simulink model "W06_8_ned"  (R2024b)
settings: Solver=ode4  StartTime=0.0  StopTime=T_run  FixedStep=Ts_ctrl  RelTol=1e-3
InitFcn:
  | if ~exist('W06_model_init','file'), addpath(fileparts(get_param('W06_8_ned','FileName'))); end, W06_model_init('W06_8_ned')
StopFcn:
  | W06_model_done('W06_8_ned')
values from neighbouring files (symbols this model uses):
  alloc_prm = [half_beam; l_bow; F_max; F_bow_max]    [W06_setup.m]
  animate = 0    [W06_bow_demo.m]    (also in W06_psi_sweep.m; W06_setup.m = 1)
  beta_c = deg2rad(current_direction)    [W06_setup.m]
  bow_on = BOW(i)    [W06_bow_demo.m]    (also in W06_setup.m = 1)
  current_speed = 0.0    (= 0)    [W06_setup.m]
  F_bow_max = 250    [W06_setup.m]
  F_max = 500    [W06_setup.m]
  F_plugin_max = 2353.53383667818    (= 2353.53383668)    [W06_setup.m]
  half_beam = 1.027135    [W06_setup.m]
  k_prop = 1000 * 0.004422 * 0.2^4    (= 0.0070752)    [W06_setup.m]
  Kb = Ki_u / Kp_u    (= 0.333333333333)    [W06_setup.m]
  Kd_psi = 200    [W06_setup.m]
  Ki_vn = 100    [W06_setup.m]
  Kp_ned = 0.4    [W06_setup.m]
  Kp_psi = 400    [W06_setup.m]
  Kp_vn = 300    [W06_setup.m]
  l_bow = 0.75    [W06_setup.m]
  stop_hold = 15    [W06_setup.m]
  task_mode = 3    [W06_setup.m]
  task_q = [ hold_north;  hold_east;  deg2rad(hold_deg) ... (first row only)    [W06_setup.m]
  Ts_ctrl = 0.05    [W06_setup.m]
  usv_p = [m_usv; Izz; Xu; Xuu; Yv; Yvv; Nr; Nrr; half_beam; l_bow]    [W06_setup.m]
  V_ned_max = v_max    (= 0.6)    [W06_setup.m]
  x0 = [0.1; 0; 0; 0; 0; psi_init]    [W06_setup.m]
libraries: slpidlib x2
settings Model: Creator=admin  LastModifiedBy=admin

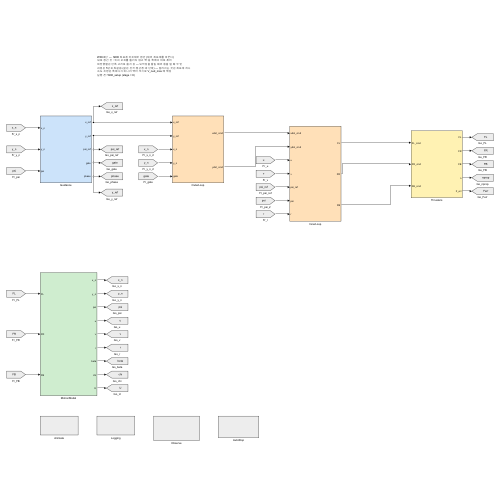
[thumbnail: Simulink's stored preview of the top-level diagram]
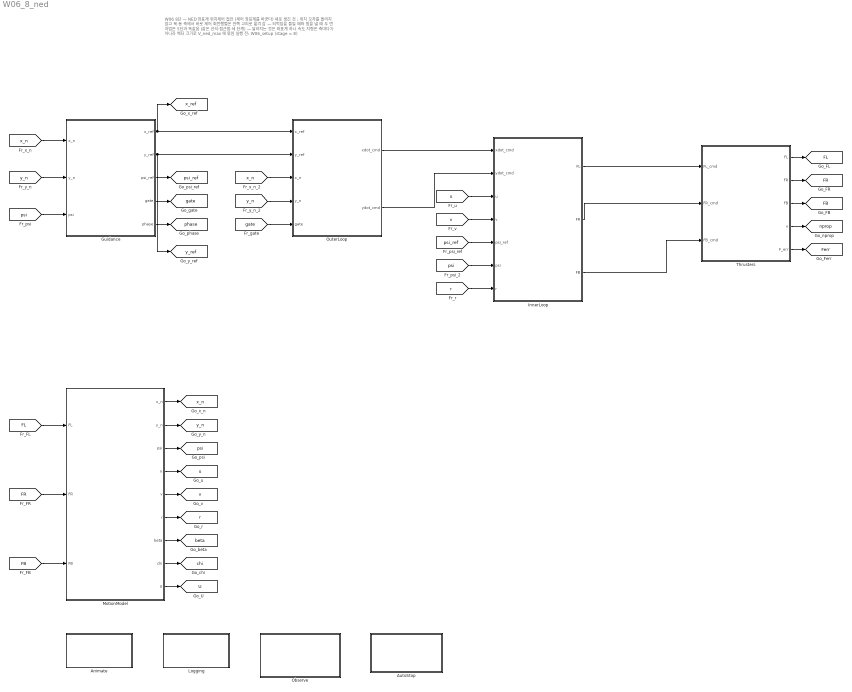
== system W06_8_ned ==
  note: W06 8단  —  NED 좌표계 위치제어 접안 (제어 좌표계를 바꾼다)
      | 새로 생긴 것 : 위치 오차를 돌리지 않고 북·동 축에서 바로 제어
      | 회전행렬은 안쪽 고리로 옮겨 감 — 되먹임을 들일 때와 힘을 낼 때 두 번
      | 과업은 5단과 똑같음 (같은 선석·접근점·세 단계) — 달라지는 것은 좌표계 하나
      | 속도 지령은 축마다가 아니라 벡터 크기로 V_ned_max 에 묶임
      | 실행 전: W06_setup (stage = 8)
  Animate : Subsystem
  AutoStop : Subsystem
  Guidance : Subsystem
  InnerLoop : Subsystem
  Logging : Subsystem
  MotionModel : Subsystem
  Observe : Subsystem
  OuterLoop : Subsystem
  Thrusters : Subsystem
  tag scope: FB=global, FL=global, FR=global, Ferr=global, U=global, beta=global, chi=global, gate=global, nprop=global, phase=global, psi=global, psi_ref=global, r=global, u=global, v=global, x_n=global, x_ref=global, y_n=global, y_ref=global
  wires:
  InnerLoop/3(FB) -> Thrusters/3(FB_cmd)
  InnerLoop/2(FR) -> Thrusters/2(FR_cmd)
  InnerLoop/1(FL) -> Thrusters/1(FL_cmd)
  OuterLoop/2(ydot_cmd) -> InnerLoop/2(ydot_cmd)
  OuterLoop/1(xdot_cmd) -> InnerLoop/1(xdot_cmd)
  Guidance/1(x_ref) -> OuterLoop/1(x_ref), [x_ref]
  Guidance/2(y_ref) -> OuterLoop/2(y_ref), [y_ref]
  Thrusters/1(FL) -> [FL]
  Thrusters/2(FR) -> [FR]
  Thrusters/4(n) -> [nprop]
  MotionModel/3(psi) -> [psi]
  Guidance/3(psi_ref) -> [psi_ref]
  MotionModel/6(r) -> [r]
  MotionModel/4(u) -> [u]
  MotionModel/5(v) -> [v]
  MotionModel/1(x_n) -> [x_n]
  MotionModel/2(y_n) -> [y_n]
  [FB] -> MotionModel/3(FB)
  [FL] -> MotionModel/1(FL)
  [FR] -> MotionModel/2(FR)
  [psi_ref] -> InnerLoop/5(psi_ref)
  [r] -> InnerLoop/7(r)
  [v] -> InnerLoop/4(v)
  [x_n] -> Guidance/1(x_n)
  [x_n] -> OuterLoop/3(x_n)
  [y_n] -> Guidance/2(y_n)
  [y_n] -> OuterLoop/4(y_n)
  Thrusters/3(FB) -> [FB]
  Thrusters/5(F_err) -> [Ferr]
  MotionModel/9(U) -> [U]
  MotionModel/7(beta) -> [beta]
  MotionModel/8(chi) -> [chi]
  Guidance/4(gate) -> [gate]
  Guidance/5(phase) -> [phase]
  [gate] -> OuterLoop/5(gate)
  [psi] -> Guidance/3(psi)
  [psi] -> InnerLoop/6(psi)
  [u] -> InnerLoop/3(u)

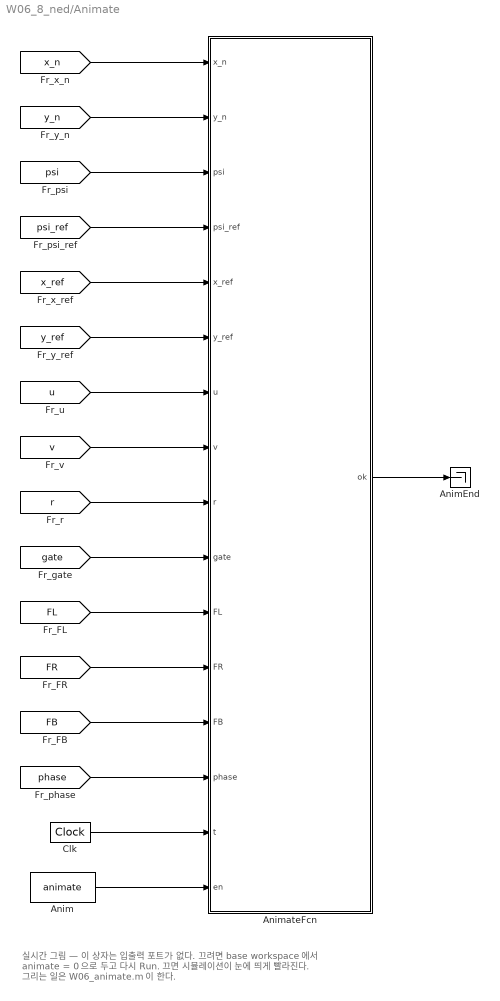
== system W06_8_ned/Animate ==
  note: 실시간 그림 — 이 상자는 입출력 포트가 없다.
      | 끄려면 base workspace 에서  animate = 0  으로 두고 다시 Run.
      | 끄면 시뮬레이션이 눈에 띄게 빨라진다.
      | 그리는 일은 W06_animate.m 이 한다.
  Anim : Constant  Value=animate
  AnimEnd : Terminator
  AnimateFcn : MATLAB Function  TreatAsAtomicUnit=on
  Clk : DigitalClock  SampleTime=Ts_ctrl
  wires:
  [x_n] -> AnimateFcn/1(x_n)
  [y_n] -> AnimateFcn/2(y_n)
  [psi] -> AnimateFcn/3(psi)
  [psi_ref] -> AnimateFcn/4(psi_ref)
  [x_ref] -> AnimateFcn/5(x_ref)
  [y_ref] -> AnimateFcn/6(y_ref)
  [u] -> AnimateFcn/7(u)
  [v] -> AnimateFcn/8(v)
  [r] -> AnimateFcn/9(r)
  [gate] -> AnimateFcn/10(gate)
  [FL] -> AnimateFcn/11(FL)
  [FR] -> AnimateFcn/12(FR)
  [FB] -> AnimateFcn/13(FB)
  [phase] -> AnimateFcn/14(phase)
  Clk/1 -> AnimateFcn/15(t)
  Anim/1 -> AnimateFcn/16(en)
  AnimateFcn/1(ok) -> AnimEnd/1

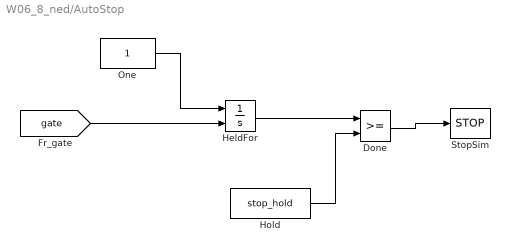
== system W06_8_ned/AutoStop ==
  Done : RelationalOperator  OutDataTypeStr=boolean  RndMeth=Simplest  InputSameDT=off
  HeldFor : Integrator  ExternalReset=level
  Hold : Constant  Value=stop_hold
  One : Constant
  StopSim : Stop
  wires:
  One/1 -> HeldFor/1
  [gate] -> HeldFor/2
  HeldFor/1 -> Done/1
  Hold/1 -> Done/2
  Done/1 -> StopSim/1

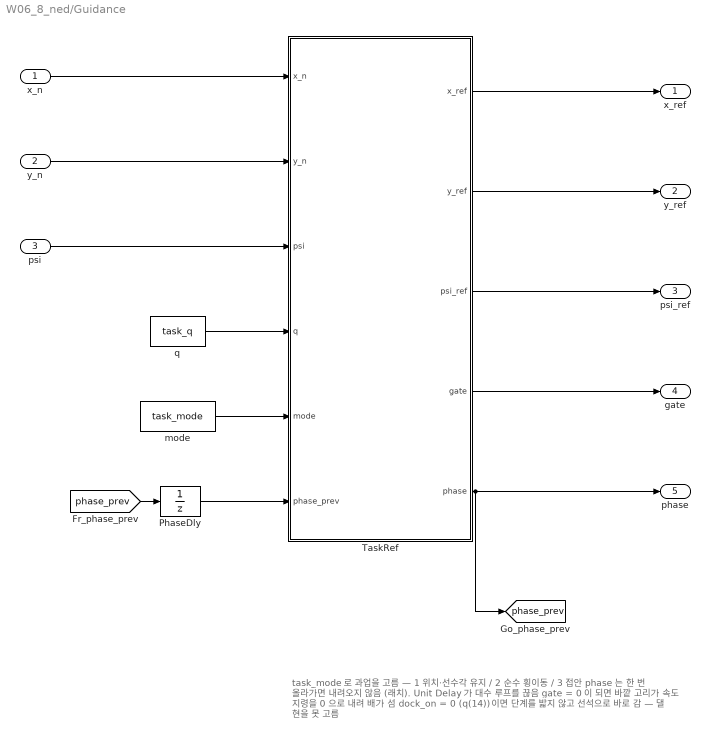
== system W06_8_ned/Guidance ==
  note: task_mode 로 과업을 고름 — 1 위치·선수각 유지 / 2 순수 횡이동 / 3 접안
      | phase 는 한 번 올라가면 내려오지 않음 (래치). Unit Delay 가 대수 루프를 끊음
      | gate = 0 이 되면 바깥 고리가 속도 지령을 0 으로 내려 배가 섬
      | dock_on = 0 (q(14)) 이면 단계를 밟지 않고 선석으로 바로 감 — 댈 현을 못 고름
  x_n : Inport
  y_n : Inport  Port=2
  psi : Inport  Port=3
  PhaseDly : UnitDelay  Description=phase 래치가 자기 자신을 입력으로 받으므로 그대로 되먹이면 대수 루프가 된다. 한 스텝 전 값을 쓰는 것 말고는 끊을 방법이 없는 자리다. 표본 간격을 고정 스텝(Ts_ctrl)과 같게 두어 연속 솔버(ode4)와 어긋나지 않는다.  SampleTime=Ts_ctrl  HasFrameUpgradeWarning=on
  TaskRef : MATLAB Function  TreatAsAtomicUnit=on
  mode : Constant  Value=task_mode
  q : Constant  Value=task_q
  x_ref : Outport
  y_ref : Outport  Port=2
  psi_ref : Outport  Port=3
  gate : Outport  Port=4
  phase : Outport  Port=5
  tag scope: phase_prev=global
  wires:
  x_n/1 -> TaskRef/1(x_n)
  y_n/1 -> TaskRef/2(y_n)
  psi/1 -> TaskRef/3(psi)
  q/1 -> TaskRef/4(q)
  mode/1 -> TaskRef/5(mode)
  PhaseDly/1 -> TaskRef/6(phase_prev)
  TaskRef/1(x_ref) -> x_ref/1
  TaskRef/2(y_ref) -> y_ref/1
  TaskRef/3(psi_ref) -> psi_ref/1
  TaskRef/4(gate) -> gate/1
  TaskRef/5(phase) -> phase/1, [phase_prev]
  [phase_prev] -> PhaseDly/1

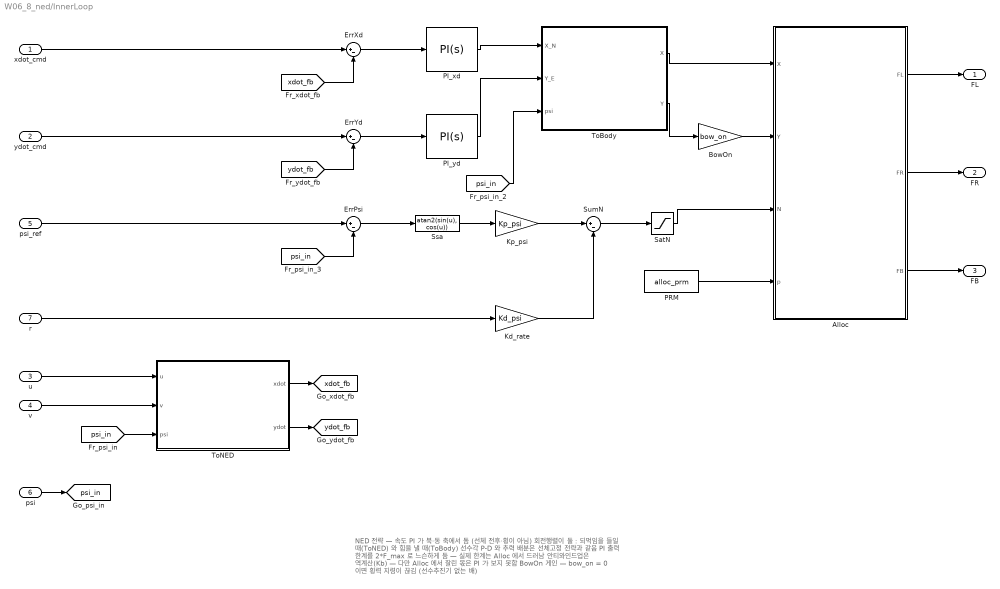
== system W06_8_ned/InnerLoop ==
  note: NED 전략 — 속도 PI 가 북·동 축에서 돔 (선체 전후·횡이 아님)
      | 회전행렬이 둘 : 되먹임을 들일 때(ToNED) 와 힘을 낼 때(ToBody)
      | 선수각 P-D 와 추력 배분은 선체고정 전략과 같음
      | PI 출력 한계를 2*F_max 로 느슨하게 둠 — 실제 한계는 Alloc 에서 드러남
      | 안티와인드업은 역계산(Kb) — 다만 Alloc 에서 잘린 몫은 PI 가 보지 못함
      | BowOn 게인 — bow_on = 0 이면 횡력 지령이 끊김 (선수추진기 없는 배)
  xdot_cmd : Inport
  ydot_cmd : Inport  Port=2
  u : Inport  Port=3
  v : Inport  Port=4
  psi_ref : Inport  Port=5
  psi : Inport  Port=6
  r : Inport  Port=7
  Alloc : MATLAB Function  TreatAsAtomicUnit=on
  BowOn : Gain  Gain=bow_on
  ErrPsi : Sum  Inputs=|+-
  ErrXd : Sum  Inputs=|+-
  ErrYd : Sum  Inputs=|+-
  Kd_rate : Gain  Gain=Kd_psi
  Kp_psi : Gain  Gain=Kp_psi
  PI_xd : slpidlib/PID Controller  Controller=PI  Form=Parallel  TimeDomain=Continuous-time  UseExternalTs=off  SampleTime=-1  IntegratorMethod=Forward Euler  FilterMethod=Forward Euler  ControllerParametersSource=internal  P=Kp_vn  I=Ki_vn  UseKiTs=off  D=0  UseExternalDerivativeSource=off  N=100  UseFilter=on  TunerSelectOption=Transfer Function Based (PID Tuner App)  InitialConditionSource=internal  InitialConditionForIntegrator=0  InitialConditionForFilter=0  DifferentiatorICPrevScaledInput=0  ExternalReset=none  TrackingMode=off  Kt=1  LimitOutput=on  SatLimitsSource=internal  UpperSaturationLimit=2*F_max  LowerSaturationLimit=-(2*F_max)  LinearizeAsGain=on  AntiWindupMode=back-calculation  Kb=Kb  LimitIntegrator=off  UpperIntegratorSaturationLimit=inf  LowerIntegratorSaturationLimit=-inf  POutMin=[]  POutMax=[]  IOutMin=[]  IOutMax=[]  DOutMin=[]  DOutMax=[]  NOutMin=[]  NOutMax=[]  SumOutMin=[]  SumOutMax=[]  SaturationOutMin=[]  SaturationOutMax=[]  PParamMin=[]  PParamMax=[]  IParamMin=[]  IParamMax=[]  DParamMin=[]  DParamMax=[]  NParamMin=[]  NParamMax=[]  KbParamMin=[]  KbParamMax=[]  KtParamMin=[]  KtParamMax=[]  KbOutMin=[]  KbOutMax=[]  KtOutMin=[]  KtOutMax=[]  IntegratorOutMin=[]  IntegratorOutMax=[]  FilterOutMin=[]  FilterOutMax=[]  SumI1OutMin=[]  SumI1OutMax=[]  SumI2OutMin=[]  SumI2OutMax=[]  SumI3OutMin=[]  SumI3OutMax=[]  SumI4OutMin=[]  SumI4OutMax=[]  SumDOutMin=[]  SumDOutMax=[]  DifferentiatorOutMin=[]  DifferentiatorOutMax=[]  FilterDiffOutCoefMin=[]  FilterDiffOutCoefMax=[]  ReciprocalOutMin=[]  ReciprocalOutMax=[]  SumDenOutMin=[]  SumDenOutMax=[]  SumNumOutMin=[]  SumNumOutMax=[]  DivideOutMin=[]  DivideOutMax=[]  UdiffTsProdOutMin=[]  UdiffTsProdOutMax=[]  NTsProdOutMin=[]  NTsProdOutMax=[]  UintegralTsProdOutMin=[]  UintegralTsProdOutMax=[]  UngainTsProdOutMin=[]  UngainTsProdOutMax=[]  ClampingZeroOutDataTypeStr=Inherit: Inherit via back propagation  ClampingZeroOutMin=[]  ClampingZeroOutMax=[]  FilterDenConstantOutDataTypeStr=Inherit: Inherit via back propagation  FilterDenConstantOutMin=[]  FilterDenConstantOutMax=[]  PCopyOutDataTypeStr=Inherit: Inherit via back propagation  PCopyOutMin=[]  PCopyOutMax=[]  NCopyOutDataTypeStr=Inherit: Inherit via back propagation  NCopyOutMin=[]  NCopyOutMax=[]  IntegratorContinuousStateAttributes=''  IntegratorStateMustResolveToSignalObject=off  IntegratorRTWStateStorageClass=Auto  FilterContinuousStateAttributes=''  FilterStateMustResolveToSignalObject=off  FilterRTWStateStorageClass=Auto  ParallelPVariant=InternalParameters  IdealPVariant=Disabled  IVariant=InternalParameters  DVariant=Disabled  IntegratorVariant=Continuous  SatVariant=Enabled  AWVariant=BackCalculation  PCopyVariant=Disabled  TRVariant=Disabled  FdbkBlocksVariant=Forward  IdealPFdbkVariant=Disabled  SatFdbkVariant=Disabled  DerivativeFilterVariant=Disabled  NVariant=Disabled  NCopyVariant=Disabled_SignalSpec  FilterICVariant=Disabled  IntegratorICVariant=InternalICs  ExternalResetVariant=Disabled  TRSumVariant=Passthrough  SumFdbkVariant=Disabled  SumVariant=Sum_PI  TsampFilterVariant=InternalTs  TsampNgainVariant=Passthrough  TsampIntegralVariant=Disabled_SignalSpec  ExternalSaturationOutDataTypeStr=Inherit: Same as second input  DerivativeSourceVariant=Disabled  PreIntVariant=InternalPreInt
  PI_yd : slpidlib/PID Controller  Controller=PI  Form=Parallel  TimeDomain=Continuous-time  UseExternalTs=off  SampleTime=-1  IntegratorMethod=Forward Euler  FilterMethod=Forward Euler  ControllerParametersSource=internal  P=Kp_vn  I=Ki_vn  UseKiTs=off  D=0  UseExternalDerivativeSource=off  N=100  UseFilter=on  TunerSelectOption=Transfer Function Based (PID Tuner App)  InitialConditionSource=internal  InitialConditionForIntegrator=0  InitialConditionForFilter=0  DifferentiatorICPrevScaledInput=0  ExternalReset=none  TrackingMode=off  Kt=1  LimitOutput=on  SatLimitsSource=internal  UpperSaturationLimit=2*F_max  LowerSaturationLimit=-(2*F_max)  LinearizeAsGain=on  AntiWindupMode=back-calculation  Kb=Kb  LimitIntegrator=off  UpperIntegratorSaturationLimit=inf  LowerIntegratorSaturationLimit=-inf  POutMin=[]  POutMax=[]  IOutMin=[]  IOutMax=[]  DOutMin=[]  DOutMax=[]  NOutMin=[]  NOutMax=[]  SumOutMin=[]  SumOutMax=[]  SaturationOutMin=[]  SaturationOutMax=[]  PParamMin=[]  PParamMax=[]  IParamMin=[]  IParamMax=[]  DParamMin=[]  DParamMax=[]  NParamMin=[]  NParamMax=[]  KbParamMin=[]  KbParamMax=[]  KtParamMin=[]  KtParamMax=[]  KbOutMin=[]  KbOutMax=[]  KtOutMin=[]  KtOutMax=[]  IntegratorOutMin=[]  IntegratorOutMax=[]  FilterOutMin=[]  FilterOutMax=[]  SumI1OutMin=[]  SumI1OutMax=[]  SumI2OutMin=[]  SumI2OutMax=[]  SumI3OutMin=[]  SumI3OutMax=[]  SumI4OutMin=[]  SumI4OutMax=[]  SumDOutMin=[]  SumDOutMax=[]  DifferentiatorOutMin=[]  DifferentiatorOutMax=[]  FilterDiffOutCoefMin=[]  FilterDiffOutCoefMax=[]  ReciprocalOutMin=[]  ReciprocalOutMax=[]  SumDenOutMin=[]  SumDenOutMax=[]  SumNumOutMin=[]  SumNumOutMax=[]  DivideOutMin=[]  DivideOutMax=[]  UdiffTsProdOutMin=[]  UdiffTsProdOutMax=[]  NTsProdOutMin=[]  NTsProdOutMax=[]  UintegralTsProdOutMin=[]  UintegralTsProdOutMax=[]  UngainTsProdOutMin=[]  UngainTsProdOutMax=[]  ClampingZeroOutDataTypeStr=Inherit: Inherit via back propagation  ClampingZeroOutMin=[]  ClampingZeroOutMax=[]  FilterDenConstantOutDataTypeStr=Inherit: Inherit via back propagation  FilterDenConstantOutMin=[]  FilterDenConstantOutMax=[]  PCopyOutDataTypeStr=Inherit: Inherit via back propagation  PCopyOutMin=[]  PCopyOutMax=[]  NCopyOutDataTypeStr=Inherit: Inherit via back propagation  NCopyOutMin=[]  NCopyOutMax=[]  IntegratorContinuousStateAttributes=''  IntegratorStateMustResolveToSignalObject=off  IntegratorRTWStateStorageClass=Auto  FilterContinuousStateAttributes=''  FilterStateMustResolveToSignalObject=off  FilterRTWStateStorageClass=Auto  ParallelPVariant=InternalParameters  IdealPVariant=Disabled  IVariant=InternalParameters  DVariant=Disabled  IntegratorVariant=Continuous  SatVariant=Enabled  AWVariant=BackCalculation  PCopyVariant=Disabled  TRVariant=Disabled  FdbkBlocksVariant=Forward  IdealPFdbkVariant=Disabled  SatFdbkVariant=Disabled  DerivativeFilterVariant=Disabled  NVariant=Disabled  NCopyVariant=Disabled_SignalSpec  FilterICVariant=Disabled  IntegratorICVariant=InternalICs  ExternalResetVariant=Disabled  TRSumVariant=Passthrough  SumFdbkVariant=Disabled  SumVariant=Sum_PI  TsampFilterVariant=InternalTs  TsampNgainVariant=Passthrough  TsampIntegralVariant=Disabled_SignalSpec  ExternalSaturationOutDataTypeStr=Inherit: Same as second input  DerivativeSourceVariant=Disabled  PreIntVariant=InternalPreInt
  PRM : Constant  Value=alloc_prm
  SatN : Saturate  UpperLimit=2*F_max*half_beam + F_bow_max*l_bow  LowerLimit=-(2*F_max*half_beam + F_bow_max*l_bow)
  Ssa : Fcn  Expr=atan2(sin(u), cos(u))
  SumN : Sum  Inputs=|+-
  ToBody : MATLAB Function  TreatAsAtomicUnit=on
  ToNED : MATLAB Function  TreatAsAtomicUnit=on
  FL : Outport
  FR : Outport  Port=2
  FB : Outport  Port=3
  tag scope: psi_in=global, xdot_fb=global, ydot_fb=global
  wires:
  ErrPsi/1 -> Ssa/1
  u/1 -> ToNED/1(u)
  v/1 -> ToNED/2(v)
  psi/1 -> [psi_in]
  [psi_in] -> ToNED/3(psi)
  [psi_in] -> ToBody/3(psi)
  [psi_in] -> ErrPsi/2
  xdot_cmd/1 -> ErrXd/1
  ydot_cmd/1 -> ErrYd/1
  ToNED/1(xdot) -> [xdot_fb]
  ToNED/2(ydot) -> [ydot_fb]
  [xdot_fb] -> ErrXd/2
  [ydot_fb] -> ErrYd/2
  ErrXd/1 -> PI_xd/1
  ErrYd/1 -> PI_yd/1
  PI_xd/1 -> ToBody/1(X_N)
  PI_yd/1 -> ToBody/2(Y_E)
  psi_ref/1 -> ErrPsi/1
  Ssa/1 -> Kp_psi/1
  r/1 -> Kd_rate/1
  Kp_psi/1 -> SumN/1
  Kd_rate/1 -> SumN/2
  SumN/1 -> SatN/1
  ToBody/1(X) -> Alloc/1(X)
  ToBody/2(Y) -> BowOn/1
  BowOn/1 -> Alloc/2(Y)
  SatN/1 -> Alloc/3(N)
  PRM/1 -> Alloc/4(p)
  Alloc/1(FL) -> FL/1
  Alloc/2(FR) -> FR/1
  Alloc/3(FB) -> FB/1

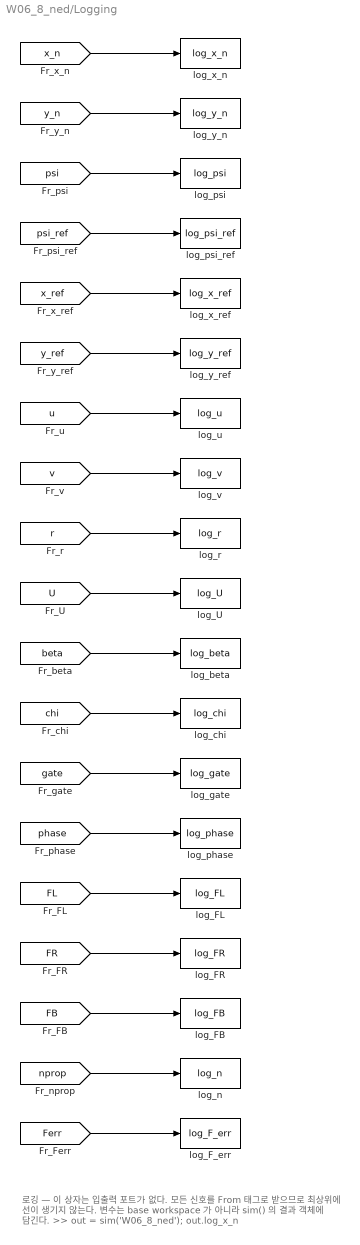
== system W06_8_ned/Logging ==
  note: 로깅 — 이 상자는 입출력 포트가 없다.
      | 모든 신호를 From 태그로 받으므로 최상위에 선이 생기지 않는다.
      | 변수는 base workspace 가 아니라 sim() 의 결과 객체에 담긴다.
      |   >> out = sim('W06_8_ned');  out.log_x_n
  log_FB : ToWorkspace  VariableName=log_FB  SaveFormat=Timeseries  SampleTime=Ts_ctrl
  log_FL : ToWorkspace  VariableName=log_FL  SaveFormat=Timeseries  SampleTime=Ts_ctrl
  log_FR : ToWorkspace  VariableName=log_FR  SaveFormat=Timeseries  SampleTime=Ts_ctrl
  log_F_err : ToWorkspace  VariableName=log_F_err  SaveFormat=Timeseries  SampleTime=Ts_ctrl
  log_U : ToWorkspace  VariableName=log_U  SaveFormat=Timeseries  SampleTime=Ts_ctrl
  log_beta : ToWorkspace  VariableName=log_beta  SaveFormat=Timeseries  SampleTime=Ts_ctrl
  log_chi : ToWorkspace  VariableName=log_chi  SaveFormat=Timeseries  SampleTime=Ts_ctrl
  log_gate : ToWorkspace  VariableName=log_gate  SaveFormat=Timeseries  SampleTime=Ts_ctrl
  log_n : ToWorkspace  VariableName=log_n  SaveFormat=Timeseries  SampleTime=Ts_ctrl
  log_phase : ToWorkspace  VariableName=log_phase  SaveFormat=Timeseries  SampleTime=Ts_ctrl
  log_psi : ToWorkspace  VariableName=log_psi  SaveFormat=Timeseries  SampleTime=Ts_ctrl
  log_psi_ref : ToWorkspace  VariableName=log_psi_ref  SaveFormat=Timeseries  SampleTime=Ts_ctrl
  log_r : ToWorkspace  VariableName=log_r  SaveFormat=Timeseries  SampleTime=Ts_ctrl
  log_u : ToWorkspace  VariableName=log_u  SaveFormat=Timeseries  SampleTime=Ts_ctrl
  log_v : ToWorkspace  VariableName=log_v  SaveFormat=Timeseries  SampleTime=Ts_ctrl
  log_x_n : ToWorkspace  VariableName=log_x_n  SaveFormat=Timeseries  SampleTime=Ts_ctrl
  log_x_ref : ToWorkspace  VariableName=log_x_ref  SaveFormat=Timeseries  SampleTime=Ts_ctrl
  log_y_n : ToWorkspace  VariableName=log_y_n  SaveFormat=Timeseries  SampleTime=Ts_ctrl
  log_y_ref : ToWorkspace  VariableName=log_y_ref  SaveFormat=Timeseries  SampleTime=Ts_ctrl
  wires:
  [x_n] -> log_x_n/1
  [y_n] -> log_y_n/1
  [psi] -> log_psi/1
  [psi_ref] -> log_psi_ref/1
  [x_ref] -> log_x_ref/1
  [y_ref] -> log_y_ref/1
  [u] -> log_u/1
  [v] -> log_v/1
  [r] -> log_r/1
  [U] -> log_U/1
  [beta] -> log_beta/1
  [chi] -> log_chi/1
  [gate] -> log_gate/1
  [phase] -> log_phase/1
  [FL] -> log_FL/1
  [FR] -> log_FR/1
  [FB] -> log_FB/1
  [nprop] -> log_n/1
  [Ferr] -> log_F_err/1

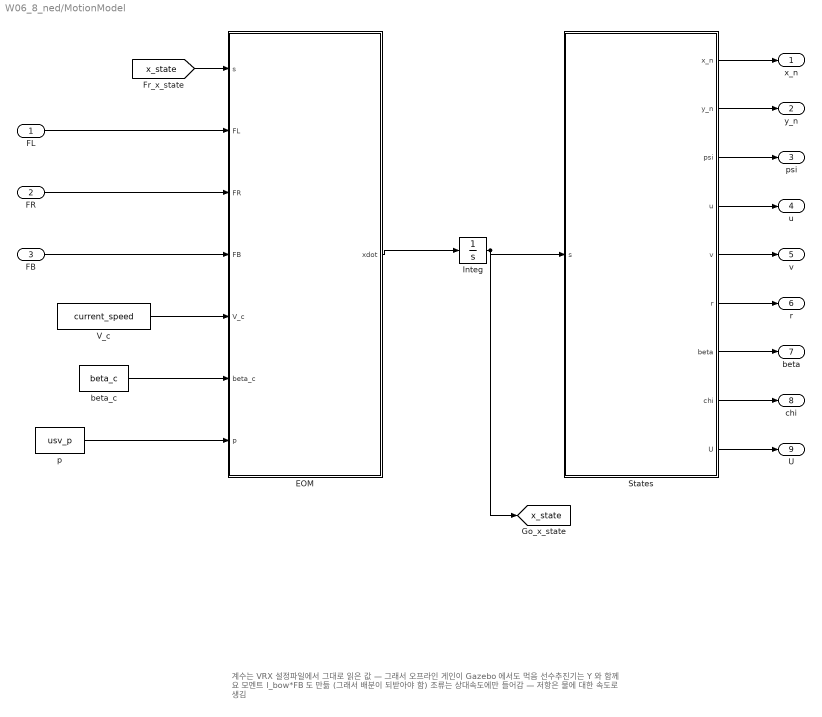
== system W06_8_ned/MotionModel ==
  note: 계수는 VRX 설정파일에서 그대로 읽은 값 — 그래서 오프라인 게인이 Gazebo 에서도 먹음
      | 선수추진기는 Y 와 함께 요 모멘트 l_bow*FB 도 만듦 (그래서 배분이 되받아야 함)
      | 조류는 상대속도에만 들어감 — 저항은 물에 대한 속도로 생김
  FL : Inport
  FR : Inport  Port=2
  FB : Inport  Port=3
  EOM : MATLAB Function  TreatAsAtomicUnit=on
  Integ : Integrator  InitialCondition=x0
  States : MATLAB Function  TreatAsAtomicUnit=on
  V_c : Constant  Value=current_speed
  beta_c : Constant  Value=beta_c
  p : Constant  Value=usv_p
  x_n : Outport
  y_n : Outport  Port=2
  psi : Outport  Port=3
  u : Outport  Port=4
  v : Outport  Port=5
  r : Outport  Port=6
  beta : Outport  Port=7
  chi : Outport  Port=8
  U : Outport  Port=9
  tag scope: x_state=global
  wires:
  FL/1 -> EOM/2(FL)
  FR/1 -> EOM/3(FR)
  FB/1 -> EOM/4(FB)
  V_c/1 -> EOM/5(V_c)
  beta_c/1 -> EOM/6(beta_c)
  p/1 -> EOM/7(p)
  EOM/1(xdot) -> Integ/1
  Integ/1 -> States/1(s), [x_state]
  [x_state] -> EOM/1(s)
  States/1(x_n) -> x_n/1
  States/2(y_n) -> y_n/1
  States/3(psi) -> psi/1
  States/4(u) -> u/1
  States/5(v) -> v/1
  States/6(r) -> r/1
  States/7(beta) -> beta/1
  States/8(chi) -> chi/1
  States/9(U) -> U/1

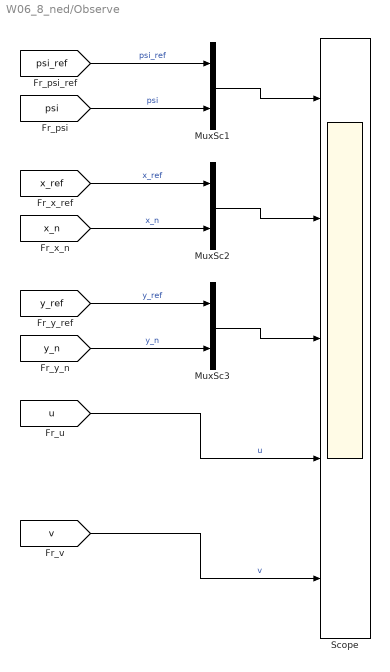
== system W06_8_ned/Observe ==
  MuxSc1 : Mux  Inputs=2
  MuxSc2 : Mux  Inputs=2
  MuxSc3 : Mux  Inputs=2
  Scope : Scope  NumInputPorts=5
  wires:
  [psi_ref] -> MuxSc1/1  "psi_ref"
  [psi] -> MuxSc1/2  "psi"
  MuxSc1/1 -> Scope/1
  [x_ref] -> MuxSc2/1  "x_ref"
  [x_n] -> MuxSc2/2  "x_n"
  MuxSc2/1 -> Scope/2
  [y_ref] -> MuxSc3/1  "y_ref"
  [y_n] -> MuxSc3/2  "y_n"
  MuxSc3/1 -> Scope/3
  [u] -> Scope/4  "u"
  [v] -> Scope/5  "v"

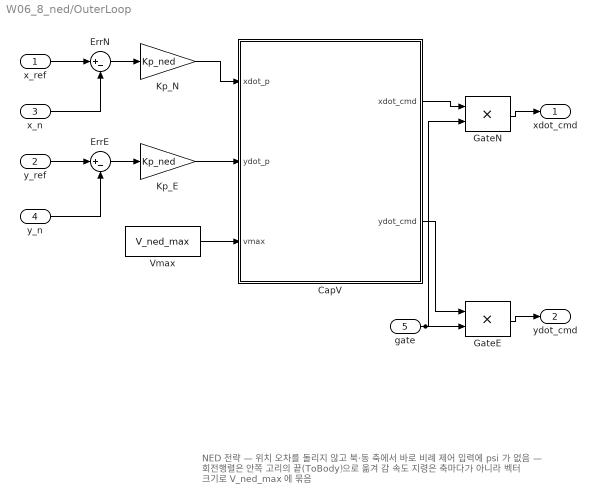
== system W06_8_ned/OuterLoop ==
  note: NED 전략 — 위치 오차를 돌리지 않고 북·동 축에서 바로 비례 제어
      | 입력에 psi 가 없음 — 회전행렬은 안쪽 고리의 끝(ToBody)으로 옮겨 감
      | 속도 지령은 축마다가 아니라 벡터 크기로 V_ned_max 에 묶음
  x_ref : Inport
  y_ref : Inport  Port=2
  x_n : Inport  Port=3
  y_n : Inport  Port=4
  gate : Inport  Port=5
  CapV : MATLAB Function  TreatAsAtomicUnit=on
  ErrE : Sum  Inputs=|+-
  ErrN : Sum  Inputs=|+-
  GateE : Product
  GateN : Product
  Kp_E : Gain  Gain=Kp_ned
  Kp_N : Gain  Gain=Kp_ned
  Vmax : Constant  Value=V_ned_max
  xdot_cmd : Outport
  ydot_cmd : Outport  Port=2
  wires:
  y_ref/1 -> ErrE/1
  x_ref/1 -> ErrN/1
  CapV/1(xdot_cmd) -> GateN/1
  x_n/1 -> ErrN/2
  ErrE/1 -> Kp_E/1
  y_n/1 -> ErrE/2
  Kp_E/1 -> CapV/2(ydot_p)
  ErrN/1 -> Kp_N/1
  Kp_N/1 -> CapV/1(xdot_p)
  Vmax/1 -> CapV/3(vmax)
  CapV/2(ydot_cmd) -> GateE/1
  gate/1 -> GateN/2, GateE/2
  GateN/1 -> xdot_cmd/1
  GateE/1 -> ydot_cmd/1

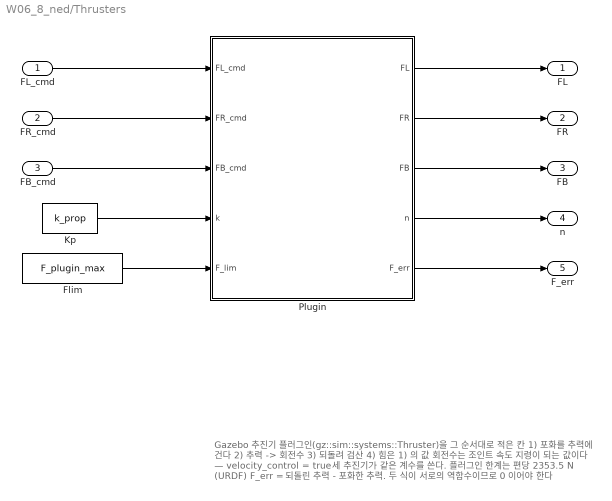
== system W06_8_ned/Thrusters ==
  note: Gazebo 추진기 플러그인(gz::sim::systems::Thruster)을 그 순서대로 적은 칸
      | 1) 포화를 추력에 건다  2) 추력 -> 회전수  3) 되돌려 검산  4) 힘은 1) 의 값
      | 회전수는 조인트 속도 지령이 되는 값이다 — velocity_control = true
      | 세 추진기가 같은 계수를 쓴다. 플러그인 한계는 편당 2353.5 N (URDF)
      | F_err = 되돌린 추력 - 포화한 추력. 두 식이 서로의 역함수이므로 0 이어야 한다
  FL_cmd : Inport
  FR_cmd : Inport  Port=2
  FB_cmd : Inport  Port=3
  Flim : Constant  Value=F_plugin_max
  Kp : Constant  Value=k_prop
  Plugin : MATLAB Function  TreatAsAtomicUnit=on
  FL : Outport
  FR : Outport  Port=2
  FB : Outport  Port=3
  n : Outport  Port=4
  F_err : Outport  Port=5
  wires:
  FL_cmd/1 -> Plugin/1(FL_cmd)
  FR_cmd/1 -> Plugin/2(FR_cmd)
  FB_cmd/1 -> Plugin/3(FB_cmd)
  Kp/1 -> Plugin/4(k)
  Flim/1 -> Plugin/5(F_lim)
  Plugin/1(FL) -> FL/1
  Plugin/2(FR) -> FR/1
  Plugin/3(FB) -> FB/1
  Plugin/4(n) -> n/1
  Plugin/5(F_err) -> F_err/1

== matlab function W06_8_ned/MotionModel/States ==
  data: s input; x_n output; y_n output; psi output; u output; v output; r output; beta output; chi output; U output
function [x_n, y_n, psi, u, v, r, beta, chi, U] = States(s)
%#codegen
%  상태벡터를 쓰기 좋은 이름으로 풀어 놓는다.
%    U    대지속력 [m/s]
%    beta 크랩각 — 뱃머리와 실제 가는 방향의 차이 [rad]
%    chi  침로 = psi + beta, 실제 가는 방향 [rad]
u = s(1);  v = s(2);  r = s(3);
x_n = s(4);  y_n = s(5);  psi = s(6);
U = sqrt(u*u + v*v);
beta = atan2(v, u);
c = psi + beta;
chi = atan2(sin(c), cos(c));

== matlab function W06_8_ned/Animate/AnimateFcn ==
  data: x_n input; y_n input; psi input; psi_ref input; x_ref input; y_ref input; u input; ok output; v input; r input; gate input; FL input; FR input; FB input; phase input; t input; en input
function ok = AnimateFcn(x_n, y_n, psi, psi_ref, x_ref, y_ref, u, v, r, gate, FL, FR, FB, phase, t, en)
%#codegen
% Live plot while the model runs. A MATLAB Function block cannot
% plot, so the drawing function is declared extrinsic: Simulink
% calls plain MATLAB instead of generating code for it.
coder.extrinsic('W06_animate');
ok = 1;
if en > 0.5
    W06_animate(x_n, y_n, psi, psi_ref, x_ref, y_ref, u, v, r, gate, FL, FR, FB, phase, t);
end

== matlab function W06_8_ned/OuterLoop/CapV ==
  data: xdot_p input; xdot_cmd output; ydot_p input; vmax input; ydot_cmd output
function [xdot_cmd, ydot_cmd] = CapV(xdot_p, ydot_p, vmax)
%#codegen
%  NED 속도 지령의 크기를 vmax 로 묶는다 (방향은 그대로).
%
%  축마다 따로 자르지 않는 까닭: 두 축을 각각 vmax 로 자르면 비스듬한
%  방향에서 크기가 vmax*sqrt(2) 가 되어 한계를 넘는다.
s = sqrt(xdot_p^2 + ydot_p^2);
if s > vmax
    xdot_cmd = xdot_p*vmax/s;
    ydot_cmd = ydot_p*vmax/s;
else
    xdot_cmd = xdot_p;
    ydot_cmd = ydot_p;
end

== matlab function W06_8_ned/Guidance/TaskRef ==
  data: x_n input; x_ref output; y_n input; psi input; q input; mode input; phase_prev input; y_ref output; psi_ref output; gate output; phase output
function [x_ref, y_ref, psi_ref, gate, phase] = TaskRef(x_n, y_n, psi, q, mode, phase_prev)
%#codegen
%  과업이 요구하는 목표 자세와 진행 단계를 내놓는다.
%
%    q(1:3)   위치유지 목표   north, east, 선수각 [rad]
%    q(4:6)   횡이동 목표     north, east, 선수각 [rad]
%    q(7:9)   접안 목표       north, east, 선수각 [rad]
%    q(10)    R_dock      접근점에 닿았다고 보는 반지름 [m]
%    q(11)    L_app       접안점에서 접근점까지의 거리 [m]
%    q(12)    berth_side  +1 이면 부두가 좌현쪽 — 접근점이 우현쪽에 생긴다
%    q(13)    R_stop      목표에 닿았다고 보는 반지름 [m]
%    q(14)    dock_on     1 이면 세 단계를 밟고, 0 이면 선석으로 바로 간다
%
%  gate = 1 이면 바깥 고리가 속도 지령을 낸다. 0 이면 멈춘다.
hx = q(1);  hy = q(2);  hpsi = q(3);
sx = q(4);  sy = q(5);  spsi = q(6);
dx = q(7);  dy = q(8);  dpsi = q(9);
Rd = q(10); La = q(11); sd = q(12); Rs = q(13);  don = q(14);
ph = phase_prev;

if mode == 1 || mode == 2
    %  한 점·한 선수각으로 가서 서 있는다. 1 과 2 는 목표만 다르다
    if mode == 1
        x_ref = hx;  y_ref = hy;  psi_ref = hpsi;
    else
        x_ref = sx;  y_ref = sy;  psi_ref = spsi;
    end
    d = sqrt((x_ref - x_n)^2 + (y_ref - y_n)^2);
    e = atan2(sin(psi_ref - psi), cos(psi_ref - psi));
    if ph < 1 && d < Rs && abs(e) < 5*pi/180
        ph = 1;                   %  도착 — 한 번 올라가면 내려오지 않는다
    end
    phase = ph;
    gate  = double(ph < 1);
else
    %  접안 — 접근점은 접안점에서 부두 반대쪽으로 L_app 만큼 떨어진 점.
    %  선수각 dpsi 로 들어가려면 접근점이 그 뒤쪽에 있어야 한다
    ax = dx - sd*La*sin(dpsi);
    ay = dy + sd*La*cos(dpsi);
    if don < 0.5
        %  단계를 나누지 않는 경우 — 목표가 처음부터 선석이다. 선수각은
        %  가는 방향으로 두므로 어느 현을 댈지 고르지 못한다
        x_ref = dx;  y_ref = dy;
        psi_ref = atan2(dy - y_n, dx - x_n);
        if sqrt((dx - x_n)^2 + (dy - y_n)^2) < Rs
            ph = 3;
        end
    elseif ph < 1
        %  1단계 — 접근점으로 간다. 선수각은 가는 방향으로 둔다 (저항이 작다)
        x_ref = ax;  y_ref = ay;
        psi_ref = atan2(ay - y_n, ax - x_n);
        if sqrt((ax - x_n)^2 + (ay - y_n)^2) < Rd
            ph = 1;
        end
    elseif ph < 2
        %  2단계 — 접근점에 머물며 선수각만 접안 선수각으로 돌린다
        x_ref = ax;  y_ref = ay;  psi_ref = dpsi;
        e = atan2(sin(dpsi - psi), cos(dpsi - psi));
        if abs(e) < 5*pi/180
            ph = 2;
        end
    else
        %  3단계 — 선수각을 지킨 채 접안점으로 밀어 넣는다
        x_ref = dx;  y_ref = dy;  psi_ref = dpsi;
        if sqrt((dx - x_n)^2 + (dy - y_n)^2) < Rs
            ph = 3;
        end
    end
    phase = ph;
    gate  = double(ph < 3);
end

== matlab function W06_8_ned/InnerLoop/ToNED ==
  data: u input; xdot output; v input; psi input; ydot output
function [xdot, ydot] = ToNED(u, v, psi)
%#codegen
%  선체고정 속도를 NED 속도로 돌린다 (논문 식 14).
%
%    xdot  북쪽 속도 [m/s],   ydot  동쪽 속도 [m/s]
xdot = u*cos(psi) - v*sin(psi);
ydot = u*sin(psi) + v*cos(psi);

== matlab function W06_8_ned/InnerLoop/ToBody ==
  data: X_N input; X output; Y_E input; psi input; Y output
function [X, Y] = ToBody(X_N, Y_E, psi)
%#codegen
%  NED 힘 지령을 선체고정 힘 지령으로 돌린다 (논문 식 16).
%
%    X  전후력 [N] — 좌·우 추진기가 낸다
%    Y  횡력   [N] — 선수추진기가 낸다
X =  X_N*cos(psi) + Y_E*sin(psi);
Y = -X_N*sin(psi) + Y_E*cos(psi);

== matlab function W06_8_ned/InnerLoop/Alloc ==
  data: X input; FL output; Y input; N input; p input; FR output; FB output
function [FL, FR, FB] = Alloc(X, Y, N, p)
%#codegen
%  추력 배분 — 요구 힘·모멘트를 세 추진기로 나눈다.
%
%    X = FL + FR                      전후력 [N]
%    Y = FB                           횡력 [N]  — 선수추진기만 낸다
%    N = (FL - FR)*b + l3*FB          요 모멘트 [N m]
%
%  p = [b; l3; Fmax; Fbmax]
%    b     half_beam   좌·우 추진기까지의 반폭 [m]
%    l3    l_bow       무게중심에서 선수추진기까지 [m]
%    Fmax  선미 추진기 추력 한계 [N],  Fbmax 선수추진기 추력 한계 [N]
%
%  선수추진기가 횡력을 내면 요 모멘트 l3*FB 가 딸려 온다. 그것을 좌·우
%  추진기가 되받아 빼야 선수각이 돌아가지 않는다 — 아래 N - l3*FB 가 그것이다.
b = p(1);  l3 = p(2);  Fmax = p(3);  Fbmax = p(4);
FB = Y;
if FB >  Fbmax, FB =  Fbmax; end
if FB < -Fbmax, FB = -Fbmax; end
%  포화된 뒤의 FB 로 모멘트를 센다 — 실제로 딸려 온 만큼만 되받는다
M  = N - l3*FB;
FL = X/2 + M/(2*b);
FR = X/2 - M/(2*b);
if FL >  Fmax, FL =  Fmax; end
if FL < -Fmax, FL = -Fmax; end
if FR >  Fmax, FR =  Fmax; end
if FR < -Fmax, FR = -Fmax; end

== matlab function W06_8_ned/Thrusters/Plugin ==
  data: FL_cmd input; FL output; FR_cmd input; FB_cmd input; k input; F_lim input; FR output; FB output; n output; F_err output
function [FL, FR, FB, n, F_err] = Plugin(FL_cmd, FR_cmd, FB_cmd, k, F_lim)
%#codegen
%  Gazebo 추진기 플러그인이 하는 일을 소스와 같은 순서로 적는다.
%    gz-sim7  src/systems/thruster/Thruster.cc

%  1) 포화 — 플러그인은 **추력에** 건다 (OnCmdThrust, :520-521)
%       thrust = clamp(cmd, cmdMin, cmdMax),  cmdMax = max_thrust_cmd
F = [FL_cmd; FR_cmd; FB_cmd];
F = max(-F_lim, min(F_lim, F));

%  2) 추력 -> 회전수 (ThrustToAngularVec, :562-584). 이 값이 조인트
%     속도 지령이 된다 — velocity_control = true (:740-756)
%       omega = sign(F*Ct)*sqrt(|F|/(rho*Ct*D^4)),  k = rho*Ct*D^4
%     Ct > 0 이므로 sign(F*Ct) = sign(F) 다
n = sign(F) .* sqrt(abs(F)/k);

%  3) 회전수 -> 추력 (AngularVelToThrust, :593-599). 플러그인에서는
%     회전수 지령 모드에만 쓰인다. 여기서는 2) 를 되돌려 맞는지 보는
%     **검산**이다 — 두 식이 서로의 역함수이므로 0 이 나와야 한다
%       F = rho*Ct*D^4 * |omega| * omega
F_chk = k * abs(n) .* n;
F_err = F_chk - F;

%  4) 링크에 가는 힘은 되돌린 값이 아니라 포화만 거친 지령이다
%     (AddWorldWrench 가 desiredThrust 를 그대로 쓴다, :770-773)
FL = F(1);
FR = F(2);
FB = F(3);

== matlab function W06_8_ned/MotionModel/EOM ==
  data: s input; xdot output; FL input; FR input; FB input; V_c input; beta_c input; p input
function xdot = EOM(s, FL, FR, FB, V_c, beta_c, p)
%#codegen
%  3자유도 운동방정식.  s = [u v r x_n y_n psi]'
%
%    조류는 상대속도에만 들어간다 — 저항은 물에 대한 속도로 생긴다
%    부가질량은 0 으로 둔다 (VRX 설정도 0 이다)
u = s(1);  v = s(2);  r = s(3);  psi = s(6);
m_s  = p(1);  Izz = p(2);
Xu   = p(3);  Xuu = p(4);
Yv   = p(5);  Yvv = p(6);
Nr   = p(7);  Nrr = p(8);
b_h  = p(9);  l3  = p(10);

%  조류를 선체좌표로 — 물에 대한 상대속도 u_r, v_r
u_c = V_c*cos(beta_c - psi);
v_c = V_c*sin(beta_c - psi);
u_r = u - u_c;
v_r = v - v_c;

%  추진기가 내는 힘과 모멘트
X = FL + FR;
Y = FB;
N = (FL - FR)*b_h + l3*FB;

%  저항 — 선형 + 제곱 (제곱항이 있어 속도가 커질수록 빨리 늘어난다)
Dx = (Xu + Xuu*abs(u_r))*u_r;
Dy = (Yv + Yvv*abs(v_r))*v_r;
Dn = (Nr + Nrr*abs(r))*r;

%  v*r, -u*r 은 좌표계가 함께 돌기 때문에 생기는 항이다
du = (X - Dx)/m_s + v*r;
dv = (Y - Dy)/m_s - u*r;
dr = (N - Dn)/Izz;

%  선체속도를 NED 로 — 이것이 위치의 미분이다
xdot = [du; dv; dr; ...
        u*cos(psi) - v*sin(psi); ...
        u*sin(psi) + v*cos(psi); ...
        r];
